simulink model "sf_mandelbrot_fixpt"  (R2025b)
settings: Solver=FixedStepDiscrete  StartTime=0.0  StopTime=inf  FixedStep=0.0005  RelTol=1e-3
StopFcn:
  | clear sf_mandel_gui;
CloseFcn:
  | sf_mandel_gui('close');
settings Model: FPTRunName=Active  ExtModeAutoUpdateStatusClock=off  Creator=The MathWorks, Inc.  LastModifiedBy=The MathWorks, Inc.
settings SolverCC: AlgebraicLoopSolver=TrustRegion  MaxZcPerStep=1.0
settings DataIOCC: LimitDataPoints=on  SaveFormat=Array  SaveOutput=off  SaveTime=off  ReturnWorkspaceOutputs=off
settings OptimizationCC: BooleanDataType=off  ReuseModelBlockBuffer=off  ExpressionDepthLimit=2147483647.0  InitFltsAndDblsToZero=on  EfficientMapNaN2IntZero=off  LifeSpan=inf  BufferReusableBoundary=off
settings DebuggingCC: UnderspecifiedInitializationDetection=Classic  MergeDetectMultiDrivingBlocksExec=none  SignalResolutionControl=TryResolveAllWithWarning  MultiTaskDSMMsg=warning  MultiTaskCondExecSysMsg=none  IntegerOverflowMsg=none  FcnCallInpInsideContextMsg=warning  UnconnectedInputMsg=warning  UnconnectedOutputMsg=warning  UnconnectedLineMsg=warning  BusObjectLabelMismatch=none  StateNameClashWarn=warning  PregeneratedLibrarySubsystemCodeDiagnostic=none  SFUnexpectedBacktrackingDiag=warning  SFNoUnconditionalDefaultTransitionDiag=warning  SFExecutionAtInitializationDiag=none  IntegerSaturationMsg=none  ArithmeticOperatorsInVariantConditions=warning
settings HardwareCC: ProdBitPerPointer=32.0  ProdBitPerSizeT=32.0  ProdBitPerPtrDiffT=32.0  ProdLargestAtomicFloat=None  ProdIntDivRoundTo=Undefined  ProdEndianess=Unspecified  ProdWordSize=32.0  ProdHWDeviceType=32-bit Generic  TargetUnknown=on
settings ModelReferenceCC: EnableRefExpFcnMdlSchedulingChecks=on  PropagateSignalLabelsOutOfModel=off
settings SFSimCC: SFSimEcho=off  SimUseLocalCustomCode=off  SimParseCustomCode=off  CustomCodeUndefinedFunction=UseInterfaceOnly
settings RTWCC: RTWUseLocalCustomCode=off  GPUComputeCapability=3.5  DLArmComputeVersion=19.05
settings CodeAppCC: StateflowObjectComments=on
settings GRTTargetCC: TargetFcnLib=ansi_tfl_tmw.mat  TargetLangStandard=C89/C90 (ANSI)  CombineOutputUpdateFcns=off  GRTInterface=on
settings ConfigComp: CovMetricSettings=dcmtr  CovSaveCumulativeToWorkspaceVar=on  CovSaveSingleToWorkspaceVar=on  CovExternalEMLEnable=off  CovSFcnEnable=off

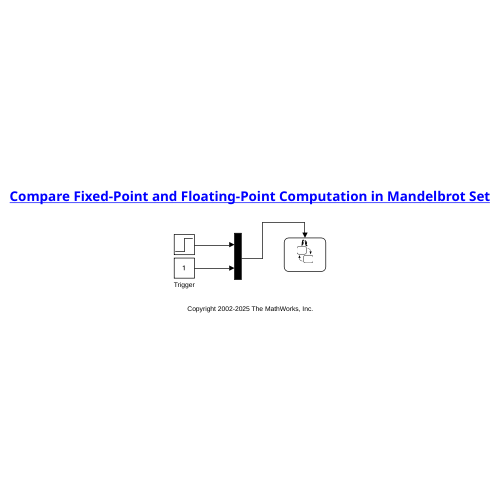
[thumbnail: Simulink's stored preview of the top-level diagram]
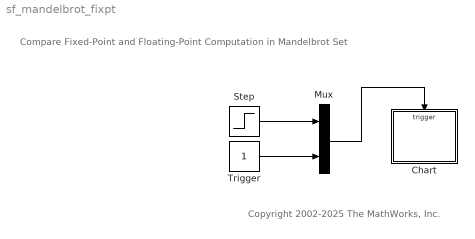
== system sf_mandelbrot_fixpt ==
  note: Copyright 2002-2025 The MathWorks, Inc.
  note: Compare Fixed-Point and Floating-Point Computation in Mandelbrot Set
  Chart : Stateflow chart  TreatAsAtomicUnit=on
  Mux : Mux  Inputs=2
  Step : Step  Time=0.1  SampleTime=0  ZeroCross=off
  Trigger : Constant
  wires:
  Trigger/1 -> Mux/2
  Step/1 -> Mux/1
  Mux/1 -> Chart/Trigger

== stateflow chart sf_mandelbrot_fixpt/Chart ==
  state ii = mandel_fix(a,b) [function]
    (default) -> (junction 28) : { a0 = fi(a, 1, 16, 13);
        |  b0 = fi(b, 1, 16, 13);
        |  c = complex(a0,b0);
        |  ii = 0;
        |  local_colors = colors;
        |  cn = fi(0+0i, 1, 32, 26); }
    (junction 30) -> (junction 28)
    (junction 33) -> (junction 30) : {
        | ii = ii + 1;
        | }
    (junction 28) -> (junction 29) : {
        | cn = c + cn .* cn;
        | }
    (junction 29) -> (junction 33) [order 1] : [ cn < 4 && ii < local_colors ]
    (junction 29) -> (junction 31) [order 2]
  state Wait
    entry:
    sf_mandel_gui('enter_wait');
  state ii = mandel_double(a0,b0) [function]
    (default) -> (junction 43) : { c = complex(a0, b0);
        |  ii = 0;
        |  local_colors = colors;
        |  cn = 0+0i; }
    (junction 41) -> (junction 43)
    (junction 44) -> (junction 41) : {
        | ii = ii + 1;
        | }
    (junction 43) -> (junction 42) : {
        | cn = c + cn .* cn;
        | }
    (junction 42) -> (junction 44) [order 1] : [ cn < 4 && ii < local_colors ]
    (junction 42) -> (junction 40) [order 2]
  (default) -> (junction 36) : {
      | coder.extrinsic('sf_mandel_gui');
      | sf_mandel_gui();
      | }
  Wait -> (junction 36) : Redraw
  (junction 36) -> (junction 45) : {
      | sf_mandel_gui('exit_wait');
      |
      | colors = sf_mandel_gui('colors');
      |
      | pix_w = sf_mandel_gui('pixel width');
      | pix_h  = sf_mandel_gui('pixel height');
      |
      | real_left = sf_mandel_gui('real left');
      | real_top = sf_mandel_gui('real top');
      | real_w   = sf_mandel_gui('real width');
      | real_h   = sf_mandel_gui('real height');
      |
      | deltax = real_w / pix_w;
      | deltay = real_h / pix_h;
      |
      | i=1;
      | y0 = real_top;
      |
      | tic();
      | }
  (junction 37) -> Wait [order 2] : {
      | toc();
      | }
  (junction 37) -> (junction 38) [order 1] : [ i <= pix_h ]
  (junction 45) -> (junction 37)
  (junction 35) -> (junction 37) [order 2] : {
      | sf_mandel_gui(i,dbl_line,fix_line);
      |
      | sf_mandel_gui('update');
      | i = i + 1;
      | y0 = y0 - deltay;
      | }
  (junction 38) -> (junction 39) : {
      | j = 1;
      | x = real_left;
      | }
  (junction 35) -> (junction 39) [order 1] : [ j <= pix_w]
  (junction 34) -> (junction 35) : {
      | j = j + 1;
      | x = x + deltax;
      | }
  (junction 39) -> (junction 32) : {
      | fix_line(j)  = mandel_fix(x,y0);
      | dbl_line(j) = mandel_double(x,y0);
      | }
  (junction 32) -> (junction 34)
  data: a function_input double; b function_input double; ii function_output int32; local_colors temporary double; c temporary fixdt(1,16,13); cn temporary fixdt(1,32,26); a0 temporary fixdt(1,16,13); b0 temporary fixdt(1,16,13); a0 function_input double; b0 function_input double; ii function_output int32; local_colors temporary double; real_left local double; real_w local double; pix_w local double; deltax local double; deltay local double; i local int32; y0 local double; j local int32; x local double; real_top local double; real_h local double; pix_h local double; colors local double; fix_line local double size=1024; dbl_line local double size=1024
  events: Start input EITHER_EDGE_EVENT; Redraw input EITHER_EDGE_EVENT
